simulink model "DRLHevIps"  (R2025b)
settings: Solver=ode23tb  StartTime=0  StopTime=stop_time+1  FixedStep=ts  RelTol=1e-3  AbsTol=1e-4
model workspace (MAT data in the model file):
  BattChrgMax : Simulink.Parameter (value not decoded)
  BattDischrgMax : Simulink.Parameter (value not decoded)
  BrkPrsMax : Simulink.Parameter (value not decoded)
  DiffRatio : Simulink.Parameter (value not decoded)
  EVSpdLmt : Simulink.Parameter (value not decoded)
  EngIdle : Simulink.Parameter (value not decoded)
  EngPwr : Simulink.Parameter (value not decoded)
  EngSpd : Simulink.Parameter (value not decoded)
  EngTrq : Simulink.Parameter (value not decoded)
  EngTrqWhl : Simulink.Parameter (value not decoded)
  GenMapEff : Simulink.Parameter (value not decoded)
  GenMapSpdIndex : Simulink.Parameter (value not decoded)
  GenMapTrqIndex : Simulink.Parameter (value not decoded)
  GenPwrMax : Simulink.Parameter (value not decoded)
  GenSpd : Simulink.Parameter (value not decoded)
  GenTrq : Simulink.Parameter (value not decoded)
  GenTrqMax : Simulink.Parameter (value not decoded)
  MotMapEff : Simulink.Parameter (value not decoded)
  MotMapSpdIndex : Simulink.Parameter (value not decoded)
  MotMapTrqIndex : Simulink.Parameter (value not decoded)
  MotPwr : Simulink.Parameter (value not decoded)
  MotSpd : Simulink.Parameter (value not decoded)
  MotTrq : Simulink.Parameter (value not decoded)
  Ndiff : Simulink.Parameter (value not decoded)
  Nr1 : Simulink.Parameter (value not decoded)
  Nr2 : Simulink.Parameter (value not decoded)
  Ns1 : Simulink.Parameter (value not decoded)
  Ns2 : Simulink.Parameter (value not decoded)
  NsysWhl : Simulink.Parameter (value not decoded)
  SOCChrgFactor : Simulink.Parameter (value not decoded)
  SOCerr : Simulink.Parameter (value not decoded)
  SOCmax : Simulink.Parameter (value not decoded)
  SOCmin : Simulink.Parameter (value not decoded)
  SOCtarget : Simulink.Parameter (value not decoded)
  SysTrqWhl : Simulink.Parameter (value not decoded)
  k : Simulink.Parameter (value not decoded)
values from neighbouring files (symbols this model uses):
  cyc_time = WLTC(:,1)    [mdlrun_time_DG.m]
  cyc_vel = WLTC(:,2)    [mdlrun_time_DG.m]
  en_actsmo = 1    [mdlrun_time_DG.m]
  en_elec = 1    [mdlrun_time_DG.m]
  en_gas = 1    [mdlrun_time_DG.m]
  en_SOCpen = 1    [mdlrun_time_DG.m]
  k_actsmo = 5e-2    (= 0.05)    [mdlrun_time_DG.m]
  k_elec = 1    [mdlrun_time_DG.m]
  k_gas = 1    [mdlrun_time_DG.m]
  k_SOCpen = 1.2    [mdlrun_time_DG.m]
  obs_max = 1e4*[0.0020, 0.0090, 0.0100, 0.0100, 8.4000, 0.0100,                0.0056, 0.1011, 2.8000,      0, 0.0001, 0.0132,                0.0740, 2.6065, 0.0339, 0.0949, 0.0117, 2.4444]    [mdlrun_time_DG.m]
  obs_min = 1e4*[0.0010, 0.0070,      0,      0, 0.8400,      0,                     0, -0.0005,     0, -2.8000,     0, -0.0032               -0.0694, -2.7092, -0.0030,    0, -0.0001, -2.7647]    [mdlrun_time_DG.m]
  Price_elec = 1    [mdlrun_time_DG.m]
  Price_gas = 7.14    [mdlrun_time_DG.m]
  rho_gas = 0.739    [mdlrun_time_DG.m]
  stop_time = cyc_time(end)    [mdlrun_time_DG.m]
  ts = 1    [mdlrun_time_DG.m]
symbols that are objects in the model workspace (value not decoded): BattChrgMax, BattDischrgMax, BrkPrsMax, DiffRatio, EngIdle, EngPwr, EngSpd, EngTrq, EngTrqWhl, EVSpdLmt, GenMapSpdIndex, GenMapTrqIndex, GenPwrMax, GenSpd, GenTrq, GenTrqMax, k, MotMapSpdIndex, MotMapTrqIndex, MotPwr, MotSpd, MotTrq, Ndiff, Nr1, Nr2, Ns1, Ns2, NsysWhl, SOCChrgFactor, SOCerr, SOCmin, SOCtarget, SysTrqWhl
undefined symbols (not defined in the file or in its folder): n_ool, T_ool
libraries: simulink x29, autolibutils x6, slpidlib x2, rllib x2, SignalEditorBlockLib x1, autolibshared x1, autolibhevctrlrcommon x1
(part 2 of 4)

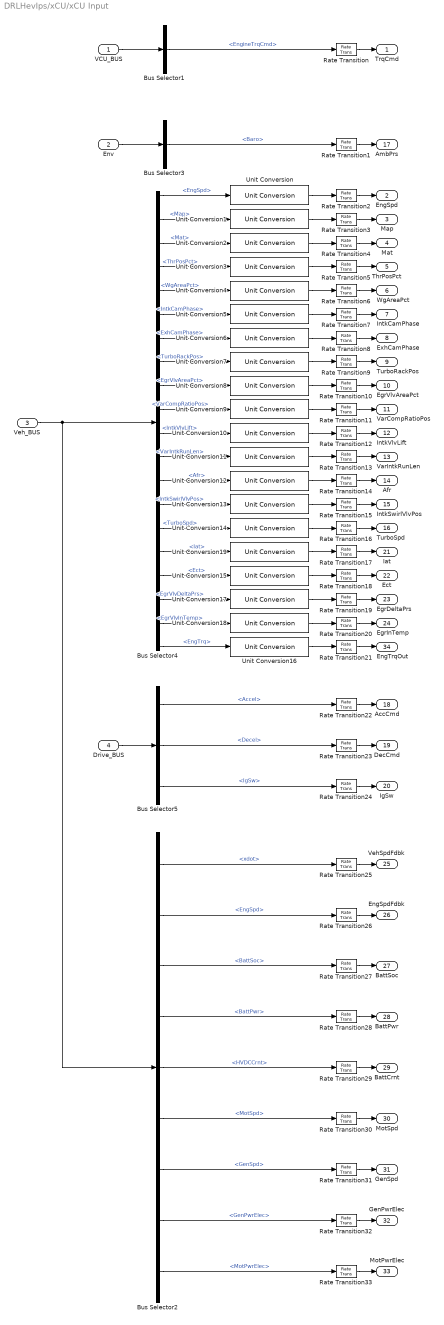
== system DRLHevIps/xCU/xCU Input ==
  VCU_BUS : Inport
  Env : Inport  Port=2
  Veh_BUS : Inport  Port=3
  Drive_BUS : Inport  Port=4
  Bus Selector1 : BusSelector  OutputSignals=EngineTrqCmd
  Bus Selector2 : BusSelector  OutputSignals=Veh.xdot,Eng.EngFdbk.EngSpd,Elec.BattSoc,Elec.BattPwr,Elec.HVDCCrnt,Veh.MotSpd,Veh.GenSpd,Elec.GenPwrElec,Elec.MotPwrElec
  Bus Selector3 : BusSelector  OutputSignals=Baro
  Bus Selector4 : BusSelector  OutputSignals=Eng.EngFdbkOut.EngSpd,Eng.EngFdbkOut.Map,Eng.EngFdbkOut.Mat,Eng.EngFdbkOut.ThrPosPct,Eng.EngFdbkOut.WgAreaPct,Eng.EngFdbkOut.IntkCamPhase,Eng.EngFdbkOut.ExhCamPhase,Eng.EngFdbkOut.TurboRackPos,Eng.EngFdbkOut.EgrVlvAreaPct,Eng.EngFdbkOut.VarCompRatioPos,Eng.EngFdbkOut.IntkVlvLift,Eng.EngFdbkOut.VarIntkRunLen,Eng.EngFdbkOut.Afr,Eng.EngFdbkOut.IntkSwirlVlvPos,Eng.EngFdbkOut.TurboSpd,Eng.EngFdbkOut.Iat,Eng.EngFdbkOut.Ect,Eng.EngFdbkOut.EgrVlvDeltaPrs,Eng.EngFdbkOut.EgrVlvInTemp,Eng.EngFdbkOut.EngTrq
  Bus Selector5 : BusSelector  OutputSignals=Info.Accel,Info.Decel,IgSw
  Rate Transition{,1..33} (34 alike) : RateTransition
  Unit Conversion{,1..19} (20 alike) : UnitConversion
  TrqCmd : Outport  VectorParamsAs1DForOutWhenUnconnected=off
  EngSpd : Outport  Port=2  VectorParamsAs1DForOutWhenUnconnected=off
  Map : Outport  Port=3  VectorParamsAs1DForOutWhenUnconnected=off
  Mat : Outport  Port=4  VectorParamsAs1DForOutWhenUnconnected=off
  ThrPosPct : Outport  Port=5  VectorParamsAs1DForOutWhenUnconnected=off
  WgAreaPct : Outport  Port=6  VectorParamsAs1DForOutWhenUnconnected=off
  IntkCamPhase : Outport  Port=7  VectorParamsAs1DForOutWhenUnconnected=off
  ExhCamPhase : Outport  Port=8  VectorParamsAs1DForOutWhenUnconnected=off
  TurboRackPos : Outport  Port=9  VectorParamsAs1DForOutWhenUnconnected=off
  EgrVlvAreaPct : Outport  Port=10  VectorParamsAs1DForOutWhenUnconnected=off
  VarCompRatioPos : Outport  Port=11  VectorParamsAs1DForOutWhenUnconnected=off
  IntkVlvLift : Outport  Port=12  VectorParamsAs1DForOutWhenUnconnected=off
  VarIntkRunLen : Outport  Port=13  VectorParamsAs1DForOutWhenUnconnected=off
  Afr : Outport  Port=14  VectorParamsAs1DForOutWhenUnconnected=off
  IntkSwirlVlvPos : Outport  Port=15  VectorParamsAs1DForOutWhenUnconnected=off
  TurboSpd : Outport  Port=16  VectorParamsAs1DForOutWhenUnconnected=off
  AmbPrs : Outport  Port=17  VectorParamsAs1DForOutWhenUnconnected=off
  AccCmd : Outport  Port=18  VectorParamsAs1DForOutWhenUnconnected=off
  DecCmd : Outport  Port=19  VectorParamsAs1DForOutWhenUnconnected=off
  IgSw : Outport  Port=20  VectorParamsAs1DForOutWhenUnconnected=off
  Iat : Outport  Port=21  VectorParamsAs1DForOutWhenUnconnected=off
  Ect : Outport  Port=22  VectorParamsAs1DForOutWhenUnconnected=off
  EgrDeltaPrs : Outport  Port=23  VectorParamsAs1DForOutWhenUnconnected=off
  EgrInTemp : Outport  Port=24  VectorParamsAs1DForOutWhenUnconnected=off
  VehSpdFdbk : Outport  Port=25  VectorParamsAs1DForOutWhenUnconnected=off
  EngSpdFdbk : Outport  Port=26  VectorParamsAs1DForOutWhenUnconnected=off
  BattSoc : Outport  Port=27  VectorParamsAs1DForOutWhenUnconnected=off
  BattPwr : Outport  Port=28  VectorParamsAs1DForOutWhenUnconnected=off
  BattCrnt : Outport  Port=29  VectorParamsAs1DForOutWhenUnconnected=off
  MotSpd : Outport  Port=30  VectorParamsAs1DForOutWhenUnconnected=off
  GenSpd : Outport  Port=31  VectorParamsAs1DForOutWhenUnconnected=off
  GenPwrElec : Outport  Port=32  VectorParamsAs1DForOutWhenUnconnected=off
  MotPwrElec : Outport  Port=33  VectorParamsAs1DForOutWhenUnconnected=off
  EngTrqOut : Outport  Port=34  Unit=N*m  VectorParamsAs1DForOutWhenUnconnected=off
  wires:
  VCU_BUS/1 -> Bus Selector1/1
  Bus Selector1/1 -> Rate Transition/1  "<EngineTrqCmd>"
  Drive_BUS/1 -> Bus Selector5/1
  Veh_BUS/1 -> Bus Selector4/1, Bus Selector2/1
  Unit Conversion6/1 -> Rate Transition8/1
  Unit Conversion1/1 -> Rate Transition3/1
  Unit Conversion14/1 -> Rate Transition16/1
  Unit Conversion12/1 -> Rate Transition14/1
  Unit Conversion2/1 -> Rate Transition4/1
  Unit Conversion13/1 -> Rate Transition15/1
  Unit Conversion7/1 -> Rate Transition9/1
  Unit Conversion4/1 -> Rate Transition6/1
  Unit Conversion3/1 -> Rate Transition5/1
  Unit Conversion5/1 -> Rate Transition7/1
  Unit Conversion10/1 -> Rate Transition12/1
  Unit Conversion11/1 -> Rate Transition13/1
  Unit Conversion/1 -> Rate Transition2/1
  Unit Conversion9/1 -> Rate Transition11/1
  Unit Conversion8/1 -> Rate Transition10/1
  Unit Conversion15/1 -> Rate Transition18/1
  Unit Conversion16/1 -> Rate Transition21/1
  Bus Selector3/1 -> Rate Transition1/1  "<Baro>"
  Env/1 -> Bus Selector3/1
  Unit Conversion17/1 -> Rate Transition19/1
  Unit Conversion18/1 -> Rate Transition20/1
  Unit Conversion19/1 -> Rate Transition17/1
  Bus Selector2/1 -> Rate Transition25/1  "<xdot>"
  Bus Selector2/2 -> Rate Transition26/1  "<EngSpd>"
  Bus Selector2/3 -> Rate Transition27/1  "<BattSoc>"
  Bus Selector2/4 -> Rate Transition28/1  "<BattPwr>"
  Bus Selector2/5 -> Rate Transition29/1  "<HVDCCrnt>"
  Bus Selector2/6 -> Rate Transition30/1  "<MotSpd>"
  Bus Selector2/7 -> Rate Transition31/1  "<GenSpd>"
  Bus Selector2/8 -> Rate Transition32/1  "<GenPwrElec>"
  Bus Selector2/9 -> Rate Transition33/1  "<MotPwrElec>"
  Bus Selector5/1 -> Rate Transition22/1  "<Accel>"
  Bus Selector5/2 -> Rate Transition23/1  "<Decel>"
  Bus Selector5/3 -> Rate Transition24/1  "<IgSw>"
  Bus Selector4/1 -> Unit Conversion/1  "<EngSpd>"
  Bus Selector4/2 -> Unit Conversion1/1  "<Map>"
  Bus Selector4/3 -> Unit Conversion2/1  "<Mat>"
  Bus Selector4/4 -> Unit Conversion3/1  "<ThrPosPct>"
  Bus Selector4/5 -> Unit Conversion4/1  "<WgAreaPct>"
  Bus Selector4/6 -> Unit Conversion5/1  "<IntkCamPhase>"
  Bus Selector4/7 -> Unit Conversion6/1  "<ExhCamPhase>"
  Bus Selector4/8 -> Unit Conversion7/1  "<TurboRackPos>"
  Bus Selector4/9 -> Unit Conversion8/1  "<EgrVlvAreaPct>"
  Bus Selector4/10 -> Unit Conversion9/1  "<VarCompRatioPos>"
  Bus Selector4/11 -> Unit Conversion10/1  "<IntkVlvLift>"
  Bus Selector4/12 -> Unit Conversion11/1  "<VarIntkRunLen>"
  Bus Selector4/13 -> Unit Conversion12/1  "<Afr>"
  Bus Selector4/14 -> Unit Conversion13/1  "<IntkSwirlVlvPos>"
  Bus Selector4/15 -> Unit Conversion14/1  "<TurboSpd>"
  Bus Selector4/16 -> Unit Conversion19/1  "<Iat>"
  Bus Selector4/17 -> Unit Conversion15/1  "<Ect>"
  Bus Selector4/18 -> Unit Conversion17/1  "<EgrVlvDeltaPrs>"
  Bus Selector4/19 -> Unit Conversion18/1  "<EgrVlvInTemp>"
  Bus Selector4/20 -> Unit Conversion16/1  "<EngTrq>"
  Rate Transition/1 -> TrqCmd/1
  Rate Transition1/1 -> AmbPrs/1
  Rate Transition15/1 -> IntkSwirlVlvPos/1
  Rate Transition11/1 -> VarCompRatioPos/1
  Rate Transition12/1 -> IntkVlvLift/1
  Rate Transition13/1 -> VarIntkRunLen/1
  Rate Transition14/1 -> Afr/1
  Rate Transition8/1 -> ExhCamPhase/1
  Rate Transition10/1 -> EgrVlvAreaPct/1
  Rate Transition17/1 -> Iat/1
  Rate Transition16/1 -> TurboSpd/1
  Rate Transition18/1 -> Ect/1
  Rate Transition9/1 -> TurboRackPos/1
  Rate Transition2/1 -> EngSpd/1
  Rate Transition3/1 -> Map/1
  Rate Transition19/1 -> EgrDeltaPrs/1
  Rate Transition20/1 -> EgrInTemp/1
  Rate Transition4/1 -> Mat/1
  Rate Transition6/1 -> WgAreaPct/1
  Rate Transition5/1 -> ThrPosPct/1
  Rate Transition7/1 -> IntkCamPhase/1
  Rate Transition21/1 -> EngTrqOut/1
  Rate Transition22/1 -> AccCmd/1
  Rate Transition23/1 -> DecCmd/1
  Rate Transition24/1 -> IgSw/1
  Rate Transition25/1 -> VehSpdFdbk/1
  Rate Transition26/1 -> EngSpdFdbk/1
  Rate Transition27/1 -> BattSoc/1
  Rate Transition28/1 -> BattPwr/1
  Rate Transition29/1 -> BattCrnt/1
  Rate Transition30/1 -> MotSpd/1
  Rate Transition31/1 -> GenSpd/1
  Rate Transition32/1 -> GenPwrElec/1
  Rate Transition33/1 -> MotPwrElec/1

== system DRLHevIps/xCU/xCU Output ==
  ThrPosPctCmd : Inport
  WgAreaPctCmd : Inport  Port=2
  InjPw : Inport  Port=3
  FuelMainSoi : Inport  Port=4
  SpkAdv : Inport  Port=5
  IntkCamPhaseCmd : Inport  Port=6
  ExhCamPhaseCmd : Inport  Port=7
  TurboRackPosCmd : Inport  Port=8
  EgrVlvAreaPctCmd : Inport  Port=9
  VarCompRatioPosCmd : Inport  Port=10
  IntkVlvLiftCmd : Inport  Port=11
  VarIntkRunLenCmd : Inport  Port=12
  ClsdLpFuelMult : Inport  Port=13
  IntkSwirlVlvPosCmd : Inport  Port=14
  TrqCmdISC : Inport  Port=15
  LoadCmd : Inport  Port=16
  EstIntkPortFlw : Inport  Port=17
  EngTrqCmd : Inport  Port=18
  GenTrqCmd : Inport  Port=19
  MotTrqCmd : Inport  Port=20
  BrakeCmd : Inport  Port=21
  Bus Creator1 : BusCreator  Inputs=4
  Bus Creator2 : BusCreator  Inputs=17
  ECU_BUS : Outport  VectorParamsAs1DForOutWhenUnconnected=off
  VCU_BUS : Outport  Port=2  VectorParamsAs1DForOutWhenUnconnected=off
  wires:
  BrakeCmd/1 -> Bus Creator1/4  "BrakeCmd"
  Bus Creator1/1 -> VCU_BUS/1  "PtCtrl"
  EngTrqCmd/1 -> Bus Creator1/1  "EngineTrqCmd"
  GenTrqCmd/1 -> Bus Creator1/2  "GenTrqCmd"
  MotTrqCmd/1 -> Bus Creator1/3  "MotTrqCmd"
  Bus Creator2/1 -> ECU_BUS/1  "EngCtrl"
  LoadCmd/1 -> Bus Creator2/16  "LoadCmd"
  TurboRackPosCmd/1 -> Bus Creator2/8  "TurboRackPosCmd"
  InjPw/1 -> Bus Creator2/3  "InjPw"
  IntkSwirlVlvPosCmd/1 -> Bus Creator2/14  "IntkSwirlVlvPosCmd"
  FuelMainSoi/1 -> Bus Creator2/4  "FuelMainSoi"
  ThrPosPctCmd/1 -> Bus Creator2/1  "ThrPosPctCmd"
  VarIntkRunLenCmd/1 -> Bus Creator2/12  "VarIntkRunLenCmd"
  TrqCmdISC/1 -> Bus Creator2/15  "TrqCmdISC"
  IntkCamPhaseCmd/1 -> Bus Creator2/6  "IntkCamPhaseCmd"
  EgrVlvAreaPctCmd/1 -> Bus Creator2/9  "EgrVlvAreaPctCmd"
  WgAreaPctCmd/1 -> Bus Creator2/2  "WgAreaPctCmd"
  SpkAdv/1 -> Bus Creator2/5  "SpkAdv"
  EstIntkPortFlw/1 -> Bus Creator2/17  "EstIntkPortFlw"
  ClsdLpFuelMult/1 -> Bus Creator2/13  "ClsdLpFuelMult"
  VarCompRatioPosCmd/1 -> Bus Creator2/10  "VarCompRatioPosCmd"
  ExhCamPhaseCmd/1 -> Bus Creator2/7  "ExhCamPhaseCmd"
  IntkVlvLiftCmd/1 -> Bus Creator2/11  "IntkVlvLiftCmd"

== system DRLHevIps/xCU/xCU/VCU ==
  AccelPed : Inport
  DecelPed : Inport  Port=2
  VehSpdFdbk : Inport  Port=3
  EngSpdFdbk : Inport  Port=4
  BattSoc : Inport  Port=5
  BattPwr : Inport  Port=6
  MotSpd : Inport  Port=7
  GenSpd : Inport  Port=8
  GenPwrElec : Inport  Port=9
  MotPwrElec : Inport  Port=10
  EngTrqOut : Inport  Port=11
  DRL_BUS : Inport  Port=12
  DRL_Based2_0 : Subsystem  VariantControl=DRLEMS
  Rule_Based : Subsystem  VariantControl=RBEMS
  Rule_Based_DataGen : Subsystem  VariantControl=RBEMSDG
  EngTrqCmd : Outport
  GenTrqCmd : Outport  Port=2
  MotTrqCmd : Outport  Port=3
  BrkCmd : Outport  Port=4
  Reward_BUS : Outport  Port=5

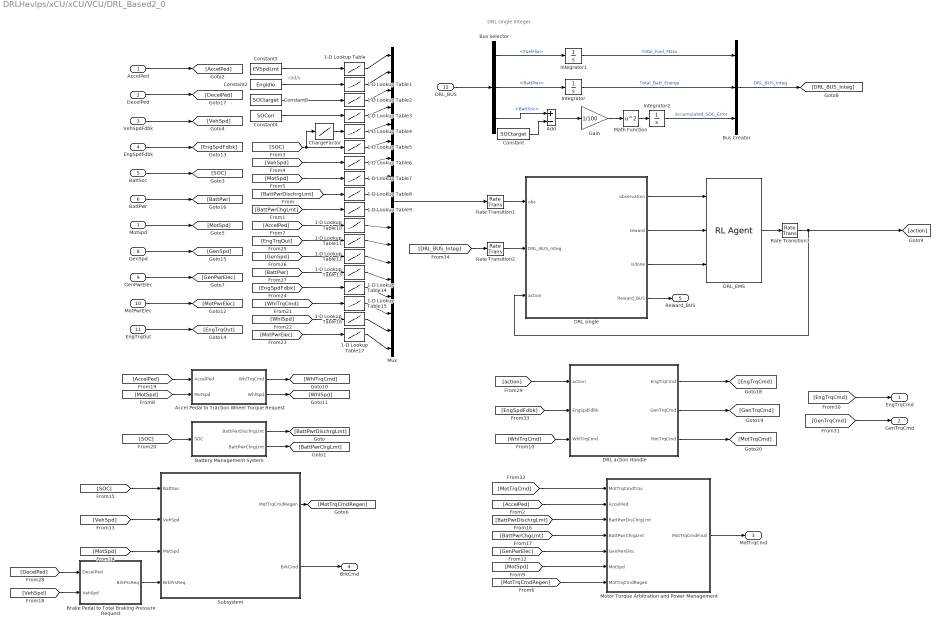
== system DRLHevIps/xCU/xCU/VCU/DRL_Based2_0 ==
  note: DRL single Integer
  note: rad/s
  AccelPed : Inport  OutDataTypeStr=double  PortDimensions=1  SampleTime=[0.01,0]
  DecelPed : Inport  Port=2  OutDataTypeStr=double  PortDimensions=1  SampleTime=[0.01,0]
  VehSpdFdbk : Inport  Port=3  OutDataTypeStr=double  PortDimensions=1  SampleTime=[0.01,0]
  EngSpdFdbk : Inport  Port=4  OutDataTypeStr=double  PortDimensions=1  SampleTime=[0.01,0]
  BattSoc : Inport  Port=5  OutDataTypeStr=double  PortDimensions=1  SampleTime=[0.01,0]
  BattPwr : Inport  Port=6  OutDataTypeStr=double  PortDimensions=1  SampleTime=[0.01,0]
  MotSpd : Inport  Port=7  OutDataTypeStr=double  PortDimensions=1  SampleTime=[0.01,0]
  GenSpd : Inport  Port=8  OutDataTypeStr=double  PortDimensions=1  SampleTime=[0.01,0]
  GenPwrElec : Inport  Port=9  OutDataTypeStr=double  PortDimensions=1  SampleTime=[0.01,0]
  MotPwrElec : Inport  Port=10  OutDataTypeStr=double  PortDimensions=1  SampleTime=[0.01,0]
  EngTrqOut : Inport  Port=11  OutDataTypeStr=double  PortDimensions=1  SampleTime=[0.01,0]
  DRL_BUS : Inport  Port=12
  1-D Lookup Table : Lookup_n-D  NumberOfTableDimensions=1  BreakpointsForDimension1=[obs_min(1), obs_max(1)]  Table=[0,1]  InternalRulePriority=Speed  RndMeth=Simplest
  1-D Lookup Table1 : Lookup_n-D  NumberOfTableDimensions=1  BreakpointsForDimension1=[obs_min(2), obs_max(2)]  Table=[0,1]  InternalRulePriority=Speed  RndMeth=Simplest
  1-D Lookup Table10 : Lookup_n-D  NumberOfTableDimensions=1  BreakpointsForDimension1=[obs_min(11), obs_max(11)]  Table=[0,1]  InternalRulePriority=Speed  RndMeth=Simplest
  1-D Lookup Table11 : Lookup_n-D  NumberOfTableDimensions=1  BreakpointsForDimension1=[obs_min(12), obs_max(12)]  Table=[0,1]  InternalRulePriority=Speed  RndMeth=Simplest
  1-D Lookup Table12 : Lookup_n-D  NumberOfTableDimensions=1  BreakpointsForDimension1=[obs_min(13), obs_max(13)]  Table=[0,1]  InternalRulePriority=Speed  RndMeth=Simplest
  1-D Lookup Table13 : Lookup_n-D  NumberOfTableDimensions=1  BreakpointsForDimension1=[obs_min(14), obs_max(14)]  Table=[0,1]  InternalRulePriority=Speed  RndMeth=Simplest
  1-D Lookup Table14 : Lookup_n-D  NumberOfTableDimensions=1  BreakpointsForDimension1=[obs_min(15), obs_max(15)]  Table=[0,1]  InternalRulePriority=Speed  RndMeth=Simplest
  1-D Lookup Table15 : Lookup_n-D  NumberOfTableDimensions=1  BreakpointsForDimension1=[obs_min(16), obs_max(16 )]  Table=[0,1]  InternalRulePriority=Speed  RndMeth=Simplest
  1-D Lookup Table16 : Lookup_n-D  NumberOfTableDimensions=1  BreakpointsForDimension1=[obs_min(17), obs_max(17)]  Table=[0,1]  InternalRulePriority=Speed  RndMeth=Simplest
  1-D Lookup Table17 : Lookup_n-D  NumberOfTableDimensions=1  BreakpointsForDimension1=[obs_min(18), obs_max(18)]  Table=[0,1]  InternalRulePriority=Speed  RndMeth=Simplest
  1-D Lookup Table2 : Lookup_n-D  NumberOfTableDimensions=1  BreakpointsForDimension1=[obs_min(3), obs_max(3)]  Table=[0,1]  InternalRulePriority=Speed  RndMeth=Simplest
  1-D Lookup Table3 : Lookup_n-D  NumberOfTableDimensions=1  BreakpointsForDimension1=[obs_min(4), obs_max(4)]  Table=[0,1]  InternalRulePriority=Speed  RndMeth=Simplest
  1-D Lookup Table4 : Lookup_n-D  NumberOfTableDimensions=1  BreakpointsForDimension1=[obs_min(5), obs_max(5)]  Table=[0,1]  InternalRulePriority=Speed  RndMeth=Simplest
  1-D Lookup Table5 : Lookup_n-D  NumberOfTableDimensions=1  BreakpointsForDimension1=[obs_min(6), obs_max(6)]  Table=[0,1]  InternalRulePriority=Speed  RndMeth=Simplest
  1-D Lookup Table6 : Lookup_n-D  NumberOfTableDimensions=1  BreakpointsForDimension1=[obs_min(7), obs_max(7)]  Table=[0,1]  InternalRulePriority=Speed  RndMeth=Simplest
  1-D Lookup Table7 : Lookup_n-D  NumberOfTableDimensions=1  BreakpointsForDimension1=[obs_min(8), obs_max(8)]  Table=[0,1]  InternalRulePriority=Speed  RndMeth=Simplest
  1-D Lookup Table8 : Lookup_n-D  NumberOfTableDimensions=1  BreakpointsForDimension1=[obs_min(9), obs_max(9)]  Table=[0,1]  InternalRulePriority=Speed  RndMeth=Simplest
  1-D Lookup Table9 : Lookup_n-D  NumberOfTableDimensions=1  BreakpointsForDimension1=[obs_min(10), obs_max(10)]  Table=[0,1]  InternalRulePriority=Speed  RndMeth=Simplest
  Accel Pedal to Traction Wheel Torque Request : Subsystem
  Add : Sum  Inputs=+-
  Battery Management System : Subsystem
  Brake Pedal to Total Braking Pressure Request : Subsystem
  Bus Creator : BusCreator  Inputs=3
  Bus Selector : BusSelector  OutputSignals=FuelFlw,BattPwr,BattSoc
  ChargeFactor : Lookup_n-D  NumberOfTableDimensions=1  BreakpointsForDimension1=[40 80]  Table=SOCChrgFactor  ExtrapMethod=Clip  UseLastTableValue=on  InternalRulePriority=Speed  RndMeth=Simplest
  Constant : Constant  Value=SOCtarget
  Constant2 : Constant  Value=EngIdle
  Constant3 : Constant  Value=EVSpdLmt
  Constant4 : Constant  Value=SOCerr
  Constant8 : Constant  Value=SOCtarget
  DRL action Handle : Subsystem
  DRL single : Subsystem
  DRL_EMS : rllib/RL Agent  Agent=DRLEMSagent  ExternalActionAsInput=off  ProvideLastAction=off  ProvideCumRwd=off  TreatAsDirectFeedthrough=on  UseStrictObservationDataTypes=off
  Gain : Gain  Gain=1/100
  Integrator : Integrator
  Integrator1 : Integrator
  Integrator2 : Integrator
  Math Function : Math  Operator=square
  Motor Torque Arbitration and Power Management : Subsystem
  Mux : Mux  Inputs=18
  Rate Transition1 : RateTransition  OutPortSampleTime=ts
  Rate Transition2 : RateTransition  OutPortSampleTime=ts
  Rate Transition3 : RateTransition  InitialCondition=-1  OutPortSampleTime=ts
  Subsystem : Subsystem
  EngTrqCmd : Outport  OutDataTypeStr=double  PortDimensions=1  SampleTime=[0.01,0]  VectorParamsAs1DForOutWhenUnconnected=off
  GenTrqCmd : Outport  Port=2  OutDataTypeStr=double  PortDimensions=1  SampleTime=[0.01,0]  VectorParamsAs1DForOutWhenUnconnected=off
  MotTrqCmd : Outport  Port=3  OutDataTypeStr=double  PortDimensions=1  SampleTime=[0.01,0]  VectorParamsAs1DForOutWhenUnconnected=off
  BrkCmd : Outport  Port=4  OutDataTypeStr=double  PortDimensions=1  SampleTime=[0.01,0]  VectorParamsAs1DForOutWhenUnconnected=off
  Reward_BUS : Outport  Port=5
  wires:
  [MotSpd] -> Accel Pedal to Traction Wheel Torque Request/2(MotSpd)
  Constant4/1 -> 1-D Lookup Table3/1
  1-D Lookup Table4/1 -> Mux/5
  Subsystem/1(" MotTrqCmdRegen") -> [MotTrqCmdRegen]
  DRL single/4(Reward_BUS) -> Reward_BUS/1
  DRL single/2(reward) -> DRL_EMS/2
  [WhlTrqCmd] -> DRL action Handle/3(WhlTrqCmd)
  1-D Lookup Table12/1 -> Mux/13
  1-D Lookup Table3/1 -> Mux/4
  1-D Lookup Table7/1 -> Mux/8
  [WhlSpd] -> 1-D Lookup Table16/1
  GenSpd/1 -> [GenSpd]
  1-D Lookup Table8/1 -> Mux/9
  1-D Lookup Table15/1 -> Mux/16
  Constant8/1 -> 1-D Lookup Table2/1
  [EngSpdFdbk] -> 1-D Lookup Table14/1
  [AccelPed] -> 1-D Lookup Table10/1
  [MotSpd] -> Motor Torque Arbitration and Power Management/6(MotSpd)
  Rate Transition2/1 -> DRL single/2(DRL_BUS_Integ)
  DRL action Handle/3(MotTrqCmd) -> [MotTrqCmd]
  [AccelPed] -> Motor Torque Arbitration and Power Management/2(AccelPed)
  1-D Lookup Table9/1 -> Mux/10
  [EngSpdFdbk] -> DRL action Handle/2(EngSpdFdbk)
  [VehSpd] -> Brake Pedal to Total Braking Pressure Request/2(VehSpd)
  BattSoc/1 -> [SOC]
  Rate Transition1/1 -> DRL single/1(obs)
  ChargeFactor/1 -> 1-D Lookup Table4/1
  [EngTrqOut] -> 1-D Lookup Table11/1
  [BattPwrChgLmt] -> 1-D Lookup Table9/1
  [GenTrqCmd] -> GenTrqCmd/1
  [GenPwrElec] -> Motor Torque Arbitration and Power Management/5(GenPwrElec)
  1-D Lookup Table2/1 -> Mux/3
  [VehSpd] -> Subsystem/2(VehSpd)
  DRL_EMS/1 -> Rate Transition3/1
  MotPwrElec/1 -> [MotPwrElec]
  Constant3/1 -> 1-D Lookup Table/1
  1-D Lookup Table17/1 -> Mux/18
  1-D Lookup Table1/1 -> Mux/2
  Motor Torque Arbitration and Power Management/1(MotTrqCmdFinal) -> MotTrqCmd/1
  Accel Pedal to Traction Wheel Torque Request/1(WhlTrqCmd) -> [WhlTrqCmd]
  1-D Lookup Table5/1 -> Mux/6
  [action] -> DRL action Handle/1(action)
  [MotTrqCmdRegen] -> Motor Torque Arbitration and Power Management/7(MotTrqCmdRegen)
  DRL action Handle/2(GenTrqCmd) -> [GenTrqCmd]
  Battery Management System/1(BattPwrDischrgLmt) -> [BattPwrDischrgLmt]
  Brake Pedal to Total Braking Pressure Request/1(BrkPrsReq) -> Subsystem/4("BrkPrsReq ")
  [EngTrqCmd] -> EngTrqCmd/1
  [MotTrqCmd] -> Motor Torque Arbitration and Power Management/1(MotTrqCmdTrac)
  MotSpd/1 -> [MotSpd]
  [BattPwrDischrgLmt] -> 1-D Lookup Table8/1
  [VehSpd] -> 1-D Lookup Table6/1
  [GenSpd] -> 1-D Lookup Table12/1
  DRL single/1(observation) -> DRL_EMS/1
  [AccelPed] -> Accel Pedal to Traction Wheel Torque Request/1(AccelPed)
  Mux/1 -> Rate Transition1/1
  1-D Lookup Table10/1 -> Mux/11
  EngSpdFdbk/1 -> [EngSpdFdbk]
  GenPwrElec/1 -> [GenPwrElec]
  [SOC] -> Battery Management System/1(SOC)
  1-D Lookup Table/1 -> Mux/1
  VehSpdFdbk/1 -> [VehSpd]
  Battery Management System/2(BattPwrChrgLmt) -> [BattPwrChgLmt]
  1-D Lookup Table11/1 -> Mux/12
  [MotPwrElec] -> 1-D Lookup Table17/1
  DRL action Handle/1(EngTrqCmd) -> [EngTrqCmd]
  EngTrqOut/1 -> [EngTrqOut]
  Accel Pedal to Traction Wheel Torque Request/2(WhlSpd) -> [WhlSpd]
  DecelPed/1 -> [DecelPed]
  [WhlTrqCmd] -> 1-D Lookup Table15/1
  [DRL_BUS_Integ] -> Rate Transition2/1
  [MotSpd] -> 1-D Lookup Table7/1
  1-D Lookup Table13/1 -> Mux/14
  [BattPwrChgLmt] -> Motor Torque Arbitration and Power Management/4("BattPwrChrgLmt ")
  AccelPed/1 -> [AccelPed]
  Subsystem/2(" BrkCmd") -> BrkCmd/1
  [SOC] -> Subsystem/1(BattSoc)
  [BattPwr] -> 1-D Lookup Table13/1
  [DecelPed] -> Brake Pedal to Total Braking Pressure Request/1(DecelPed)
  1-D Lookup Table14/1 -> Mux/15
  BattPwr/1 -> [BattPwr]
  [MotSpd] -> Subsystem/3(MotSpd)
  Constant2/1 -> 1-D Lookup Table1/1
  DRL single/3(isdone) -> DRL_EMS/3
  1-D Lookup Table6/1 -> Mux/7
  [SOC] -> 1-D Lookup Table5/1, ChargeFactor/1
  1-D Lookup Table16/1 -> Mux/17
  [BattPwrDischrgLmt] -> Motor Torque Arbitration and Power Management/3(BattPwrDisChrgLmt)
  Rate Transition3/1 -> [action], DRL single/3(action)
  Gain/1 -> Math Function/1
  Bus Creator/1 -> [DRL_BUS_Integ]  "DRL_BUS_Integ"
  Integrator2/1 -> Bus Creator/3  "Accumulated_SOC_Error"
  Integrator/1 -> Bus Creator/2  "Total_Batt_Energy"
  Integrator1/1 -> Bus Creator/1  "Total_Fuel_Mass"
  Math Function/1 -> Integrator2/1
  Bus Selector/1 -> Integrator1/1  "<FuelFlw>"
  Bus Selector/2 -> Integrator/1  "<BattPwr>"
  Add/1 -> Gain/1
  Bus Selector/3 -> Add/1  "<BattSoc>"
  DRL_BUS/1 -> Bus Selector/1
  Constant/1 -> Add/2

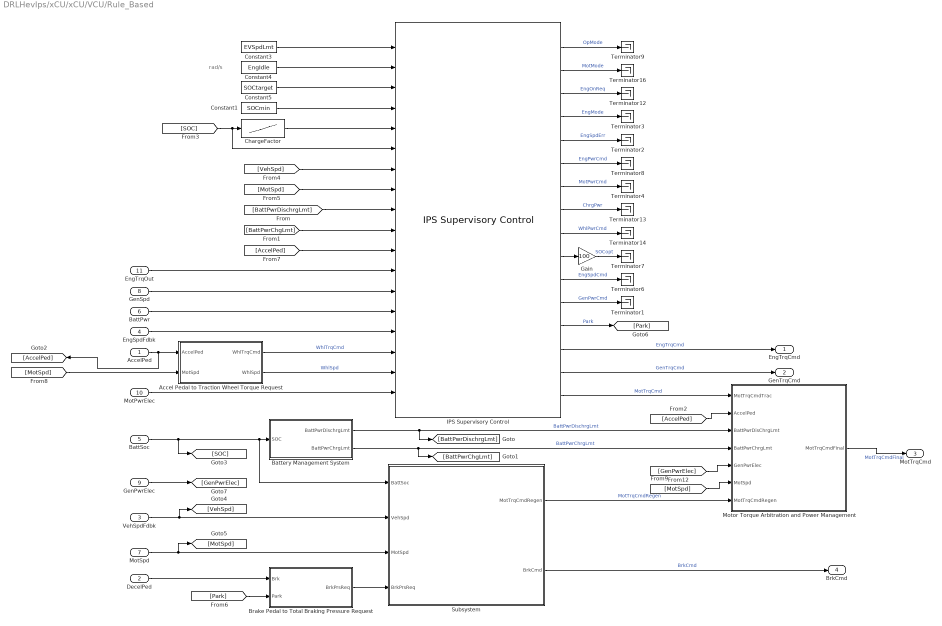
== system DRLHevIps/xCU/xCU/VCU/Rule_Based ==
  note: rad/s
  AccelPed : Inport  OutDataTypeStr=double  PortDimensions=1  SampleTime=[0.01,0]
  DecelPed : Inport  Port=2  OutDataTypeStr=double  PortDimensions=1  SampleTime=[0.01,0]
  VehSpdFdbk : Inport  Port=3  OutDataTypeStr=double  PortDimensions=1  SampleTime=[0.01,0]
  EngSpdFdbk : Inport  Port=4  OutDataTypeStr=double  PortDimensions=1  SampleTime=[0.01,0]
  BattSoc : Inport  Port=5  OutDataTypeStr=double  PortDimensions=1  SampleTime=[0.01,0]
  BattPwr : Inport  Port=6  OutDataTypeStr=double  PortDimensions=1  SampleTime=[0.01,0]
  MotSpd : Inport  Port=7  OutDataTypeStr=double  PortDimensions=1  SampleTime=[0.01,0]
  GenSpd : Inport  Port=8  OutDataTypeStr=double  PortDimensions=1  SampleTime=[0.01,0]
  GenPwrElec : Inport  Port=9  OutDataTypeStr=double  PortDimensions=1  SampleTime=[0.01,0]
  MotPwrElec : Inport  Port=10  OutDataTypeStr=double  PortDimensions=1  SampleTime=[0.01,0]
  EngTrqOut : Inport  Port=11  OutDataTypeStr=double  PortDimensions=1  SampleTime=[0.01,0]
  Accel Pedal to Traction Wheel Torque Request : Subsystem
  Battery Management System : Subsystem
  Brake Pedal to Total Braking Pressure Request : Subsystem
  ChargeFactor : Lookup_n-D  NumberOfTableDimensions=1  BreakpointsForDimension1=[40 80]  Table=SOCChrgFactor  ExtrapMethod=Clip  UseLastTableValue=on  InternalRulePriority=Speed  RndMeth=Simplest
  Constant1 : Constant  Value=SOCmin
  Constant3 : Constant  Value=EVSpdLmt
  Constant4 : Constant  Value=EngIdle
  Constant5 : Constant  Value=SOCtarget
  Gain : Gain  Gain=100
  IPS Supervisory Control : autolibhevctrlrcommon/IPS Supervisory Control  aMode=1
  Motor Torque Arbitration and Power Management : Subsystem
  Subsystem : Subsystem
  Terminator{1..4,6..9,12..14,16} (12 alike) : Terminator
  EngTrqCmd : Outport  OutDataTypeStr=double  PortDimensions=1  SampleTime=[0.01,0]  VectorParamsAs1DForOutWhenUnconnected=off
  GenTrqCmd : Outport  Port=2  OutDataTypeStr=double  PortDimensions=1  SampleTime=[0.01,0]  VectorParamsAs1DForOutWhenUnconnected=off
  MotTrqCmd : Outport  Port=3  OutDataTypeStr=double  PortDimensions=1  SampleTime=[0.01,0]  VectorParamsAs1DForOutWhenUnconnected=off
  BrkCmd : Outport  Port=4  OutDataTypeStr=double  PortDimensions=1  SampleTime=[0.01,0]  VectorParamsAs1DForOutWhenUnconnected=off
  wires:
  Gain/1 -> Terminator7/1  "SOCopt"
  Accel Pedal to Traction Wheel Torque Request/1(WhlTrqCmd) -> IPS Supervisory Control/16  "WhlTrqCmd"
  BattPwr/1 -> IPS Supervisory Control/14
  Subsystem/1(" MotTrqCmdRegen") -> Motor Torque Arbitration and Power Management/7(MotTrqCmdRegen)  "MotTrqCmdRegen"
  AccelPed/1 -> Accel Pedal to Traction Wheel Torque Request/1(AccelPed), [AccelPed]
  IPS Supervisory Control/12 -> Terminator1/1  "GenPwrCmd"
  IPS Supervisory Control/3 -> Terminator12/1  "EngOnReq"
  Brake Pedal to Total Braking Pressure Request/1(BrkPrsReq) -> Subsystem/4("BrkPrsReq ")
  IPS Supervisory Control/9 -> Terminator14/1  "WhlPwrCmd"
  [MotSpd] -> IPS Supervisory Control/8
  IPS Supervisory Control/14 -> EngTrqCmd/1  "EngTrqCmd"
  VehSpdFdbk/1 -> Subsystem/2(VehSpd), [VehSpd]
  MotSpd/1 -> Subsystem/3(MotSpd), [MotSpd]
  IPS Supervisory Control/1 -> Terminator9/1  "OpMode"
  IPS Supervisory Control/10 -> Gain/1
  [MotSpd] -> Accel Pedal to Traction Wheel Torque Request/2(MotSpd)
  EngSpdFdbk/1 -> IPS Supervisory Control/15
  [GenPwrElec] -> Motor Torque Arbitration and Power Management/5(GenPwrElec)
  Constant1/1 -> IPS Supervisory Control/4
  ChargeFactor/1 -> IPS Supervisory Control/5
  IPS Supervisory Control/2 -> Terminator16/1  "MotMode"
  IPS Supervisory Control/16 -> Motor Torque Arbitration and Power Management/1(MotTrqCmdTrac)  "MotTrqCmd"
  [Park] -> Brake Pedal to Total Braking Pressure Request/2(Park)
  [BattPwrDischrgLmt] -> IPS Supervisory Control/9
  [BattPwrChgLmt] -> IPS Supervisory Control/10
  [SOC] -> IPS Supervisory Control/6, ChargeFactor/1
  IPS Supervisory Control/8 -> Terminator13/1  "ChrgPwr"
  Accel Pedal to Traction Wheel Torque Request/2(WhlSpd) -> IPS Supervisory Control/17  "WhlSpd"
  Constant3/1 -> IPS Supervisory Control/1
  IPS Supervisory Control/6 -> Terminator8/1  "EngPwrCmd"
  Battery Management System/1(BattPwrDischrgLmt) -> Motor Torque Arbitration and Power Management/3(BattPwrDisChrgLmt), [BattPwrDischrgLmt]  "BattPwrDischrgLmt"
  Battery Management System/2(BattPwrChrgLmt) -> [BattPwrChgLmt], Motor Torque Arbitration and Power Management/4("BattPwrChrgLmt ")  "BattPwrChrgLmt"
  Motor Torque Arbitration and Power Management/1(MotTrqCmdFinal) -> MotTrqCmd/1  "MotTrqCmdFinal"
  Constant4/1 -> IPS Supervisory Control/2
  DecelPed/1 -> Brake Pedal to Total Braking Pressure Request/1(Brk)
  BattSoc/1 -> [SOC], Subsystem/1(BattSoc), Battery Management System/1(SOC)
  [AccelPed] -> IPS Supervisory Control/11
  IPS Supervisory Control/5 -> Terminator2/1  "EngSpdErr"
  GenSpd/1 -> IPS Supervisory Control/13
  GenPwrElec/1 -> [GenPwrElec]
  IPS Supervisory Control/4 -> Terminator3/1  "EngMode"
  IPS Supervisory Control/7 -> Terminator4/1  "MotPwrCmd"
  [VehSpd] -> IPS Supervisory Control/7
  MotPwrElec/1 -> IPS Supervisory Control/18
  Subsystem/2(" BrkCmd") -> BrkCmd/1  "BrkCmd"
  [AccelPed] -> Motor Torque Arbitration and Power Management/2(AccelPed)
  IPS Supervisory Control/15 -> GenTrqCmd/1  "GenTrqCmd"
  [MotSpd] -> Motor Torque Arbitration and Power Management/6(MotSpd)
  IPS Supervisory Control/11 -> Terminator6/1  "EngSpdCmd"
  Constant5/1 -> IPS Supervisory Control/3
  EngTrqOut/1 -> IPS Supervisory Control/12
  IPS Supervisory Control/13 -> [Park]  "Park"

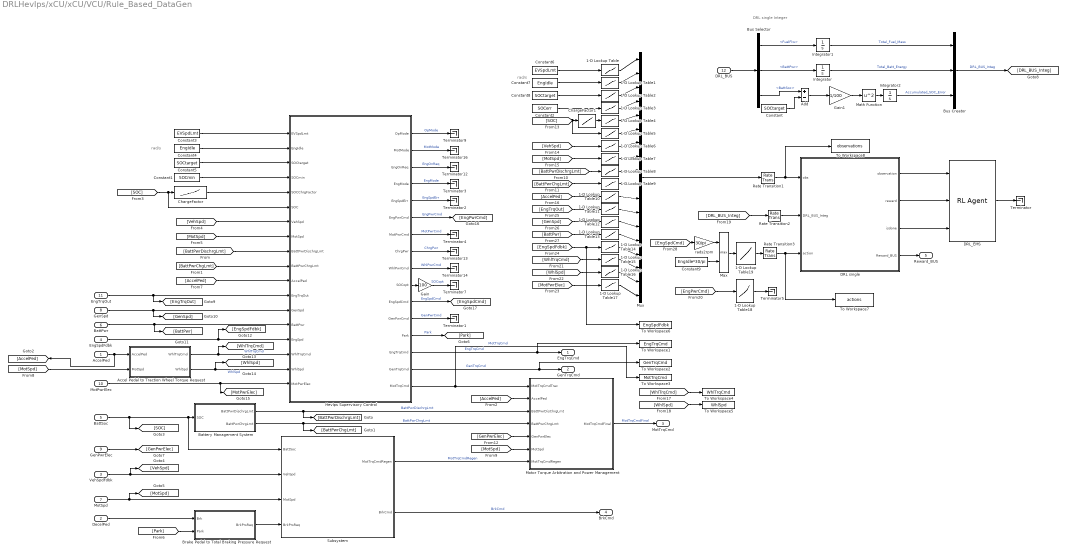
== system DRLHevIps/xCU/xCU/VCU/Rule_Based_DataGen ==
  note: rad/s
  note: rad/s
  note: DRL single Integer
  AccelPed : Inport  OutDataTypeStr=double  PortDimensions=1  SampleTime=[0.01,0]
  DecelPed : Inport  Port=2  OutDataTypeStr=double  PortDimensions=1  SampleTime=[0.01,0]
  VehSpdFdbk : Inport  Port=3  OutDataTypeStr=double  PortDimensions=1  SampleTime=[0.01,0]
  EngSpdFdbk : Inport  Port=4  OutDataTypeStr=double  PortDimensions=1  SampleTime=[0.01,0]
  BattSoc : Inport  Port=5  OutDataTypeStr=double  PortDimensions=1  SampleTime=[0.01,0]
  BattPwr : Inport  Port=6  OutDataTypeStr=double  PortDimensions=1  SampleTime=[0.01,0]
  MotSpd : Inport  Port=7  OutDataTypeStr=double  PortDimensions=1  SampleTime=[0.01,0]
  GenSpd : Inport  Port=8  OutDataTypeStr=double  PortDimensions=1  SampleTime=[0.01,0]
  GenPwrElec : Inport  Port=9  OutDataTypeStr=double  PortDimensions=1  SampleTime=[0.01,0]
  MotPwrElec : Inport  Port=10  OutDataTypeStr=double  PortDimensions=1  SampleTime=[0.01,0]
  EngTrqOut : Inport  Port=11  OutDataTypeStr=double  PortDimensions=1  SampleTime=[0.01,0]
  DRL_BUS : Inport  Port=12
  1-D Lookup Table : Lookup_n-D  NumberOfTableDimensions=1  BreakpointsForDimension1=[obs_min(1), obs_max(1)]  Table=[0,1]  InternalRulePriority=Speed  RndMeth=Simplest
  1-D Lookup Table1 : Lookup_n-D  NumberOfTableDimensions=1  BreakpointsForDimension1=[obs_min(2), obs_max(2)]  Table=[0,1]  InternalRulePriority=Speed  RndMeth=Simplest
  1-D Lookup Table10 : Lookup_n-D  NumberOfTableDimensions=1  BreakpointsForDimension1=[obs_min(11), obs_max(11)]  Table=[0,1]  InternalRulePriority=Speed  RndMeth=Simplest
  1-D Lookup Table11 : Lookup_n-D  NumberOfTableDimensions=1  BreakpointsForDimension1=[obs_min(12), obs_max(12)]  Table=[0,1]  InternalRulePriority=Speed  RndMeth=Simplest
  1-D Lookup Table12 : Lookup_n-D  NumberOfTableDimensions=1  BreakpointsForDimension1=[obs_min(13), obs_max(13)]  Table=[0,1]  InternalRulePriority=Speed  RndMeth=Simplest
  1-D Lookup Table13 : Lookup_n-D  NumberOfTableDimensions=1  BreakpointsForDimension1=[obs_min(14), obs_max(14)]  Table=[0,1]  InternalRulePriority=Speed  RndMeth=Simplest
  1-D Lookup Table14 : Lookup_n-D  NumberOfTableDimensions=1  BreakpointsForDimension1=[obs_min(15), obs_max(15)]  Table=[0,1]  InternalRulePriority=Speed  RndMeth=Simplest
  1-D Lookup Table15 : Lookup_n-D  NumberOfTableDimensions=1  BreakpointsForDimension1=[obs_min(16), obs_max(16 )]  Table=[0,1]  InternalRulePriority=Speed  RndMeth=Simplest
  1-D Lookup Table16 : Lookup_n-D  NumberOfTableDimensions=1  BreakpointsForDimension1=[obs_min(17), obs_max(17)]  Table=[0,1]  InternalRulePriority=Speed  RndMeth=Simplest
  1-D Lookup Table17 : Lookup_n-D  NumberOfTableDimensions=1  BreakpointsForDimension1=[obs_min(18), obs_max(18)]  Table=[0,1]  InternalRulePriority=Speed  RndMeth=Simplest
  1-D Lookup Table18 : Lookup_n-D  NumberOfTableDimensions=1  BreakpointsForDimension1=[0, max(EngPwr(1,1:15))]  Table=[-1, 1]  ExtrapMethod=Clip  UseLastTableValue=on  InternalRulePriority=Speed  RndMeth=Simplest
  1-D Lookup Table19 : Lookup_n-D  NumberOfTableDimensions=1  BreakpointsForDimension1=[n_ool(1), n_ool(end)]  Table=[-1, 1]  ExtrapMethod=Clip  UseLastTableValue=on  InternalRulePriority=Speed  RndMeth=Simplest
  1-D Lookup Table2 : Lookup_n-D  NumberOfTableDimensions=1  BreakpointsForDimension1=[obs_min(3), obs_max(3)]  Table=[0,1]  InternalRulePriority=Speed  RndMeth=Simplest
  1-D Lookup Table3 : Lookup_n-D  NumberOfTableDimensions=1  BreakpointsForDimension1=[obs_min(4), obs_max(4)]  Table=[0,1]  InternalRulePriority=Speed  RndMeth=Simplest
  1-D Lookup Table4 : Lookup_n-D  NumberOfTableDimensions=1  BreakpointsForDimension1=[obs_min(5), obs_max(5)]  Table=[0,1]  InternalRulePriority=Speed  RndMeth=Simplest
  1-D Lookup Table5 : Lookup_n-D  NumberOfTableDimensions=1  BreakpointsForDimension1=[obs_min(6), obs_max(6)]  Table=[0,1]  InternalRulePriority=Speed  RndMeth=Simplest
  1-D Lookup Table6 : Lookup_n-D  NumberOfTableDimensions=1  BreakpointsForDimension1=[obs_min(7), obs_max(7)]  Table=[0,1]  InternalRulePriority=Speed  RndMeth=Simplest
  1-D Lookup Table7 : Lookup_n-D  NumberOfTableDimensions=1  BreakpointsForDimension1=[obs_min(8), obs_max(8)]  Table=[0,1]  InternalRulePriority=Speed  RndMeth=Simplest
  1-D Lookup Table8 : Lookup_n-D  NumberOfTableDimensions=1  BreakpointsForDimension1=[obs_min(9), obs_max(9)]  Table=[0,1]  InternalRulePriority=Speed  RndMeth=Simplest
  1-D Lookup Table9 : Lookup_n-D  NumberOfTableDimensions=1  BreakpointsForDimension1=[obs_min(10), obs_max(10)]  Table=[0,1]  InternalRulePriority=Speed  RndMeth=Simplest
  Accel Pedal to Traction Wheel Torque Request : Subsystem
  Add : Sum  Inputs=+-
  Battery Management System : Subsystem
  Brake Pedal to Total Braking Pressure Request : Subsystem
  Bus Creator : BusCreator  Inputs=3
  Bus Selector : BusSelector  OutputSignals=FuelFlw,BattPwr,BattSoc
  ChargeFactor : Lookup_n-D  NumberOfTableDimensions=1  BreakpointsForDimension1=[40 80]  Table=SOCChrgFactor  ExtrapMethod=Clip  UseLastTableValue=on  InternalRulePriority=Speed  RndMeth=Simplest
  ChargeFactor1 : Lookup_n-D  NumberOfTableDimensions=1  BreakpointsForDimension1=[40 80]  Table=SOCChrgFactor  ExtrapMethod=Clip  UseLastTableValue=on  InternalRulePriority=Speed  RndMeth=Simplest
  Constant : Constant  Value=SOCtarget
  Constant1 : Constant  Value=SOCmin
  Constant2 : Constant  Value=SOCerr
  Constant3 : Constant  Value=EVSpdLmt
  Constant4 : Constant  Value=EngIdle
  Constant5 : Constant  Value=SOCtarget
  Constant6 : Constant  Value=EVSpdLmt
  Constant7 : Constant  Value=EngIdle
  Constant8 : Constant  Value=SOCtarget
  Constant9 : Constant  Value=EngIdle*30/pi
  DRL single : Subsystem
  DRL_EMS : rllib/RL Agent  Agent=DRLEMSagent  ExternalActionAsInput=off  ProvideLastAction=off  ProvideCumRwd=off  TreatAsDirectFeedthrough=on  UseStrictObservationDataTypes=off
  Gain : Gain  Gain=100
  Gain1 : Gain  Gain=1/100
  HevIps Supervisory Control : Stateflow chart  TreatAsAtomicUnit=on
  Integrator : Integrator
  Integrator1 : Integrator
  Integrator2 : Integrator
  Math Function : Math  Operator=square
  Max : MinMax  Function=max  Inputs=2
  Motor Torque Arbitration and Power Management : Subsystem
  Mux : Mux  Inputs=18
  Rate Transition1 : RateTransition  OutPortSampleTime=ts
  Rate Transition2 : RateTransition  OutPortSampleTime=ts
  Rate Transition3 : RateTransition  InitialCondition=-1  OutPortSampleTime=ts
  Subsystem : Subsystem
  Terminator{,1..5,7,9,12..14,16} (12 alike) : Terminator
  To Workspace1 : ToWorkspace  VariableName=EngTrqCmd  SampleTime=-1
  To Workspace2 : ToWorkspace  VariableName=GenTrqCmd  SampleTime=-1
  To Workspace3 : ToWorkspace  VariableName=MotTrqCmd  SampleTime=-1
  To Workspace4 : ToWorkspace  VariableName=WhlTrqCmd  SampleTime=-1
  To Workspace5 : ToWorkspace  VariableName=WhlSpd  SampleTime=-1
  To Workspace6 : ToWorkspace  VariableName=EngSpdFdbk  SampleTime=-1
  To Workspace7 : ToWorkspace  VariableName=actions  SampleTime=-1
  To Workspace8 : ToWorkspace  VariableName=observations  SampleTime=-1
  rads2rpm : Gain  Gain=30/pi
  EngTrqCmd : Outport  OutDataTypeStr=double  PortDimensions=1  SampleTime=[0.01,0]  VectorParamsAs1DForOutWhenUnconnected=off
  GenTrqCmd : Outport  Port=2  OutDataTypeStr=double  PortDimensions=1  SampleTime=[0.01,0]  VectorParamsAs1DForOutWhenUnconnected=off
  MotTrqCmd : Outport  Port=3  OutDataTypeStr=double  PortDimensions=1  SampleTime=[0.01,0]  VectorParamsAs1DForOutWhenUnconnected=off
  BrkCmd : Outport  Port=4  OutDataTypeStr=double  PortDimensions=1  SampleTime=[0.01,0]  VectorParamsAs1DForOutWhenUnconnected=off
  Reward_BUS : Outport  Port=5
  wires:
  [SOC] -> 1-D Lookup Table5/1, ChargeFactor1/1
  1-D Lookup Table14/1 -> Mux/15
  Constant8/1 -> 1-D Lookup Table2/1
  1-D Lookup Table10/1 -> Mux/11
  1-D Lookup Table15/1 -> Mux/16
  1-D Lookup Table17/1 -> Mux/18
  1-D Lookup Table12/1 -> Mux/13
  1-D Lookup Table9/1 -> Mux/10
  1-D Lookup Table2/1 -> Mux/3
  1-D Lookup Table6/1 -> Mux/7
  1-D Lookup Table7/1 -> Mux/8
  [EngTrqOut] -> 1-D Lookup Table11/1
  1-D Lookup Table/1 -> Mux/1
  [BattPwrDischrgLmt] -> 1-D Lookup Table8/1
  ChargeFactor1/1 -> 1-D Lookup Table4/1
  [GenSpd] -> 1-D Lookup Table12/1
  1-D Lookup Table1/1 -> Mux/2
  Constant2/1 -> 1-D Lookup Table3/1
  1-D Lookup Table11/1 -> Mux/12
  1-D Lookup Table16/1 -> Mux/17
  [MotPwrElec] -> 1-D Lookup Table17/1
  [BattPwr] -> 1-D Lookup Table13/1
  Constant6/1 -> 1-D Lookup Table/1
  [EngSpdFdbk] -> To Workspace6/1, 1-D Lookup Table14/1
  [WhlSpd] -> 1-D Lookup Table16/1
  1-D Lookup Table4/1 -> Mux/5
  1-D Lookup Table3/1 -> Mux/4
  1-D Lookup Table8/1 -> Mux/9
  [BattPwrChgLmt] -> 1-D Lookup Table9/1
  Constant7/1 -> 1-D Lookup Table1/1
  1-D Lookup Table13/1 -> Mux/14
  [VehSpd] -> 1-D Lookup Table6/1
  [AccelPed] -> 1-D Lookup Table10/1
  [WhlTrqCmd] -> 1-D Lookup Table15/1
  1-D Lookup Table5/1 -> Mux/6
  [MotSpd] -> 1-D Lookup Table7/1
  HevIps Supervisory Control/5(EngSpdErr) -> Terminator2/1  "EngSpdErr"
  Gain/1 -> Terminator7/1  "SOCopt"
  HevIps Supervisory Control/16(MotTrqCmd) -> To Workspace3/1, Motor Torque Arbitration and Power Management/1(MotTrqCmdTrac)  "MotTrqCmd"
  MotPwrElec/1 -> HevIps Supervisory Control/18(MotPwrElec), [MotPwrElec]
  EngSpdFdbk/1 -> HevIps Supervisory Control/15(EngSpd), [EngSpdFdbk]
  HevIps Supervisory Control/1(OpMode) -> Terminator9/1  "OpMode"
  Subsystem/1(" MotTrqCmdRegen") -> Motor Torque Arbitration and Power Management/7(MotTrqCmdRegen)  "MotTrqCmdRegen"
  Constant5/1 -> HevIps Supervisory Control/3(SOCtarget)
  DecelPed/1 -> Brake Pedal to Total Braking Pressure Request/1(Brk)
  VehSpdFdbk/1 -> Subsystem/2(VehSpd), [VehSpd]
  HevIps Supervisory Control/9(WhlPwrCmd) -> Terminator14/1  "WhlPwrCmd"
  HevIps Supervisory Control/8(ChrgPwr) -> Terminator13/1  "ChrgPwr"
  Subsystem/2(" BrkCmd") -> BrkCmd/1  "BrkCmd"
  Accel Pedal to Traction Wheel Torque Request/2(WhlSpd) -> HevIps Supervisory Control/17(WhlSpd), [WhlSpd]  "WhlSpd"
  [BattPwrDischrgLmt] -> HevIps Supervisory Control/9(BattPwrDischrgLmt)
  Brake Pedal to Total Braking Pressure Request/1(BrkPrsReq) -> Subsystem/4("BrkPrsReq ")
  HevIps Supervisory Control/4(EngMode) -> Terminator3/1  "EngMode"
  [GenPwrElec] -> Motor Torque Arbitration and Power Management/5(GenPwrElec)
  [SOC] -> HevIps Supervisory Control/6(SOC), ChargeFactor/1
  HevIps Supervisory Control/6(EngPwrCmd) -> [EngPwrCmd]  "EngPwrCmd"
  HevIps Supervisory Control/14(EngTrqCmd) -> To Workspace1/1, EngTrqCmd/1  "EngTrqCmd"
  HevIps Supervisory Control/2(MotMode) -> Terminator16/1  "MotMode"
  BattPwr/1 -> HevIps Supervisory Control/14(BattPwr), [BattPwr]
  EngTrqOut/1 -> HevIps Supervisory Control/12(EngTrqOut), [EngTrqOut]
  HevIps Supervisory Control/10(SOCopt) -> Gain/1
  HevIps Supervisory Control/15(GenTrqCmd) -> To Workspace2/1, GenTrqCmd/1  "GenTrqCmd"
  BattSoc/1 -> [SOC], Subsystem/1(BattSoc), Battery Management System/1(SOC)
  GenSpd/1 -> HevIps Supervisory Control/13(GenSpd), [GenSpd]
  AccelPed/1 -> Accel Pedal to Traction Wheel Torque Request/1(AccelPed), [AccelPed]
  [VehSpd] -> HevIps Supervisory Control/7(VehSpd)
  [MotSpd] -> Accel Pedal to Traction Wheel Torque Request/2(MotSpd)
  [AccelPed] -> Motor Torque Arbitration and Power Management/2(AccelPed)
  HevIps Supervisory Control/3(EngOnReq) -> Terminator12/1  "EngOnReq"
  [Park] -> Brake Pedal to Total Braking Pressure Request/2(Park)
  MotSpd/1 -> Subsystem/3(MotSpd), [MotSpd]
  Motor Torque Arbitration and Power Management/1(MotTrqCmdFinal) -> MotTrqCmd/1  "MotTrqCmdFinal"
  Battery Management System/2(BattPwrChrgLmt) -> [BattPwrChgLmt], Motor Torque Arbitration and Power Management/4("BattPwrChrgLmt ")  "BattPwrChrgLmt"
  Constant4/1 -> HevIps Supervisory Control/2(EngIdle)
  [AccelPed] -> HevIps Supervisory Control/11(AccelPed)
  Battery Management System/1(BattPwrDischrgLmt) -> Motor Torque Arbitration and Power Management/3(BattPwrDisChrgLmt), [BattPwrDischrgLmt]  "BattPwrDischrgLmt"
  Constant1/1 -> HevIps Supervisory Control/4(SOCmin)
  HevIps Supervisory Control/11(EngSpdCmd) -> [EngSpdCmd]  "EngSpdCmd"
  HevIps Supervisory Control/7(MotPwrCmd) -> Terminator4/1  "MotPwrCmd"
  HevIps Supervisory Control/12(GenPwrCmd) -> Terminator1/1  "GenPwrCmd"
  Accel Pedal to Traction Wheel Torque Request/1(WhlTrqCmd) -> HevIps Supervisory Control/16(WhlTrqCmd), [WhlTrqCmd]  "WhlTrqCmd"
  [MotSpd] -> HevIps Supervisory Control/8(MotSpd)
  ChargeFactor/1 -> HevIps Supervisory Control/5(SOCChrgFactor)
  Constant3/1 -> HevIps Supervisory Control/1(EVSpdLmt)
  [BattPwrChgLmt] -> HevIps Supervisory Control/10(BattPwrChrgLmt)
  [MotSpd] -> Motor Torque Arbitration and Power Management/6(MotSpd)
  GenPwrElec/1 -> [GenPwrElec]
  HevIps Supervisory Control/13(Park) -> [Park]  "Park"
  [WhlTrqCmd] -> To Workspace4/1
  [WhlSpd] -> To Workspace5/1
  DRL_EMS/1 -> Terminator/1
  DRL single/2(reward) -> DRL_EMS/2
  Mux/1 -> Rate Transition1/1
  DRL single/1(observation) -> DRL_EMS/1
  DRL single/4(Reward_BUS) -> Reward_BUS/1
  DRL single/3(isdone) -> DRL_EMS/3
  [DRL_BUS_Integ] -> Rate Transition2/1
  Rate Transition2/1 -> DRL single/2(DRL_BUS_Integ)
  Rate Transition1/1 -> To Workspace8/1, DRL single/1(obs)
  1-D Lookup Table19/1 -> Rate Transition3/1
  [EngPwrCmd] -> 1-D Lookup Table18/1
  Rate Transition3/1 -> To Workspace7/1, DRL single/3(action)
  1-D Lookup Table18/1 -> Terminator5/1
  [EngSpdCmd] -> rads2rpm/1
  Max/1 -> 1-D Lookup Table19/1
  rads2rpm/1 -> Max/1
  Constant9/1 -> Max/2
  Constant/1 -> Add/2
  Integrator2/1 -> Bus Creator/3  "Accumulated_SOC_Error"
  Math Function/1 -> Integrator2/1
  Bus Selector/1 -> Integrator1/1  "<FuelFlw>"
  Gain1/1 -> Math Function/1
  Integrator/1 -> Bus Creator/2  "Total_Batt_Energy"
  Bus Creator/1 -> [DRL_BUS_Integ]  "DRL_BUS_Integ"
  Add/1 -> Gain1/1
  Integrator1/1 -> Bus Creator/1  "Total_Fuel_Mass"
  DRL_BUS/1 -> Bus Selector/1
  Bus Selector/2 -> Integrator/1  "<BattPwr>"
  Bus Selector/3 -> Add/1  "<BattSoc>"

== system DRLHevIps/xCU/xCU/VCU/DRL_Based2_0/Accel Pedal to Traction Wheel Torque Request ==
  AccelPed : Inport
  MotSpd : Inport  Port=2
  MaxSysTrqWhlVsWhlSpd : Lookup_n-D  NumberOfTableDimensions=1  BreakpointsForDimension1=NsysWhl  Table=SysTrqWhl  ExtrapMethod=Clip  UseLastTableValue=on  InternalRulePriority=Speed  OutDataTypeStr=Inherit: Inherit from 'Table data'  RndMeth=Simplest
  MotSpdToWhlSpd : Gain  Gain=1/(Nr2/Ns2)/Ndiff
  Product1 : Product
  rads_to_rpm : Gain  Gain=30/pi
  WhlTrqCmd : Outport  VectorParamsAs1DForOutWhenUnconnected=off
  WhlSpd : Outport  Port=2  VectorParamsAs1DForOutWhenUnconnected=off
  wires:
  AccelPed/1 -> Product1/1
  MaxSysTrqWhlVsWhlSpd/1 -> Product1/2
  MotSpd/1 -> MotSpdToWhlSpd/1
  Product1/1 -> WhlTrqCmd/1
  MotSpdToWhlSpd/1 -> WhlSpd/1, rads_to_rpm/1
  rads_to_rpm/1 -> MaxSysTrqWhlVsWhlSpd/1

== system DRLHevIps/xCU/xCU/VCU/DRL_Based2_0/Battery Management System ==
  note: Limit battery charge / discharge power based on SOC
  SOC : Inport
  ChrgLmt : Lookup_n-D  NumberOfTableDimensions=1  BreakpointsForDimension1=[0:10:100]  Table=[1 1 1 1 1 1 1 1 0.7 0.35 0]  ExtrapMethod=Clip  UseLastTableValue=on  InternalRulePriority=Speed  RndMeth=Simplest
  DischrgLmt : Lookup_n-D  NumberOfTableDimensions=1  BreakpointsForDimension1=[0:10:100]  Table=[0 0.35 0.7 1 1 1 1 1 1 1 1]  ExtrapMethod=Clip  UseLastTableValue=on  InternalRulePriority=Speed  RndMeth=Simplest
  MaxChrg : Constant  Value=BattChrgMax
  MaxDischrg : Constant  Value=BattDischrgMax
  Product : Product
  Product1 : Product
  BattPwrDischrgLmt : Outport  VectorParamsAs1DForOutWhenUnconnected=off
  BattPwrChrgLmt : Outport  Port=2  VectorParamsAs1DForOutWhenUnconnected=off
  wires:
  DischrgLmt/1 -> Product/1
  ChrgLmt/1 -> Product1/1
  Product1/1 -> BattPwrChrgLmt/1
  Product/1 -> BattPwrDischrgLmt/1
  MaxDischrg/1 -> Product/2
  MaxChrg/1 -> Product1/2
  SOC/1 -> ChrgLmt/1, DischrgLmt/1

== system DRLHevIps/xCU/xCU/VCU/DRL_Based2_0/Brake Pedal to Total Braking Pressure Request ==
  DecelPed : Inport
  VehSpd : Inport  Port=2
  Constant : Constant  Value=BrkPrsMax
  Constant1 : Constant  Value=0.5
  Product1 : Product
  Switch : Switch  Criteria=u2 > Threshold  SaturateOnIntegerOverflow=off  InputSameDT=off
  BrkPrsReq : Outport  VectorParamsAs1DForOutWhenUnconnected=off
  wires:
  DecelPed/1 -> Switch/1
  VehSpd/1 -> Switch/2
  Constant1/1 -> Switch/3
  Switch/1 -> Product1/1
  Product1/1 -> BrkPrsReq/1
  Constant/1 -> Product1/2
